simulink model "modello_es_2"  (R2024b)
settings: Solver=VariableStepAuto  StartTime=0.0  StopTime=T  RelTol=1e-3
values from neighbouring files (symbols this model uses):
  b = b_values(i)    [es_2_main.m]
libraries: robotmobilelib x1
settings Model: Creator=feder  LastModifiedBy=feder

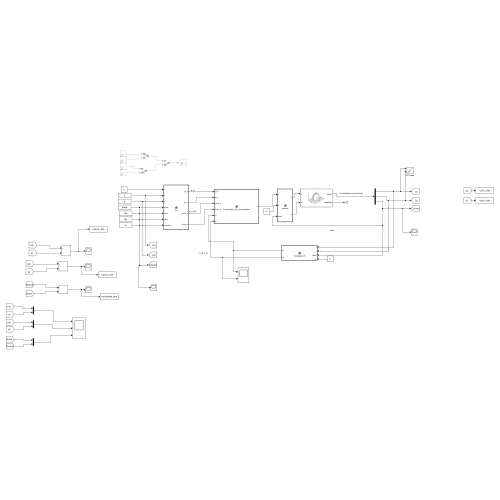
[thumbnail: Simulink's stored preview of the top-level diagram]
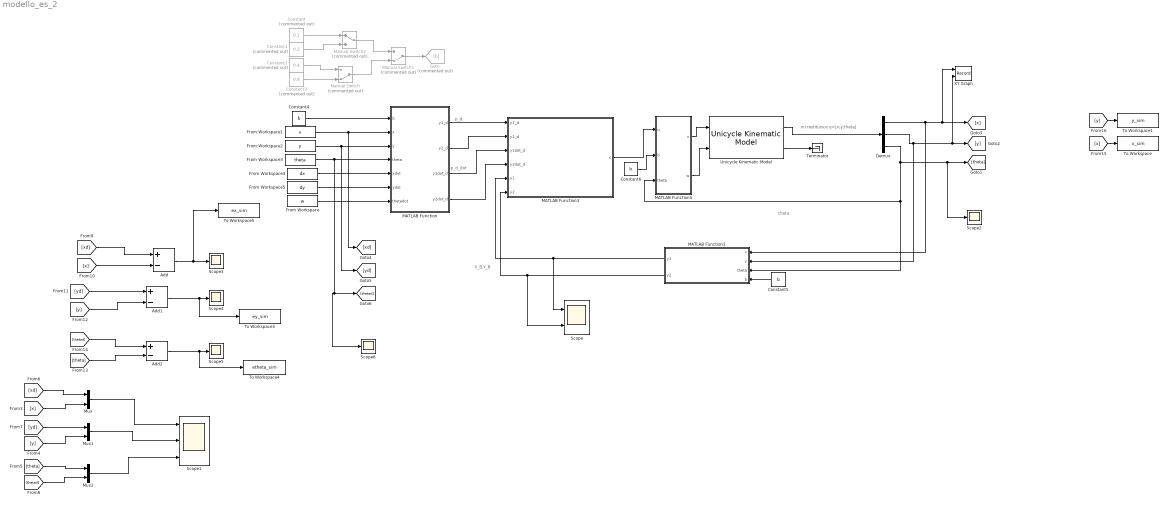
== system modello_es_2 ==
  note: theta
  note: X_B,Y_B
  note: p_d_dot
  note: p_d
  note: mi restituisce q=[x;y;theta]
  Add : Sum  Inputs=+-
  Add1 : Sum  Inputs=+-
  Add2 : Sum  Inputs=+-
  Constant : Constant  Commented=on  Value=0.1
  Constant1 : Constant  Commented=on  Value=0.2
  Constant2 : Constant  Commented=on  Value=0.4
  Constant3 : Constant  Commented=on  Value=0.8
  Constant4 : Constant  Value=b
  Constant5 : Constant  Value=b
  Constant6 : Constant  Value=b
  Demux : Demux  Outputs=3
  From Workspace : FromWorkspace  VariableName=w
  From Workspace1 : FromWorkspace  VariableName=x
  From Workspace2 : FromWorkspace  VariableName=y
  From Workspace3 : FromWorkspace  VariableName=theta
  From Workspace4 : FromWorkspace  VariableName=dx
  From Workspace5 : FromWorkspace  VariableName=dy
  Goto : Goto  Commented=on  GotoTag=b
  MATLAB Function : MATLAB Function  TreatAsAtomicUnit=on
  MATLAB Function2 : MATLAB Function  TreatAsAtomicUnit=on
  MATLAB Function3 : MATLAB Function  TreatAsAtomicUnit=on
  MATLAB Function5 : MATLAB Function  TreatAsAtomicUnit=on
  Manual Switch : ManualSwitch  Commented=on  CurrentSetting=0
  Manual Switch1 : ManualSwitch  Commented=on  CurrentSetting=0
  Manual Switch2 : ManualSwitch  Commented=on
  Mux : Mux  Inputs=2
  Mux1 : Mux  Inputs=2
  Mux2 : Mux  Inputs=2
  Scope : Scope  NumInputPorts=2
  Scope1 : Scope  NumInputPorts=3
  Scope{2..6} (5 alike) : Scope
  Terminator : Terminator
  To Workspace : ToWorkspace  VariableName=x_sim  SaveFormat=Timeseries  SampleTime=-1
  To Workspace1 : ToWorkspace  VariableName=y_sim  SaveFormat=Timeseries  SampleTime=-1
  To Workspace3 : ToWorkspace  VariableName=ey_sim  SaveFormat=Timeseries  SampleTime=-1
  To Workspace4 : ToWorkspace  VariableName=etheta_sim  SaveFormat=Timeseries  SampleTime=-1
  To Workspace5 : ToWorkspace  VariableName=ex_sim  SaveFormat=Timeseries  SampleTime=-1
  Unicycle Kinematic Model : robotmobilelib/Unicycle Kinematic Model  VehicleInputs=Vehicle Speed & Heading Angular Velocity  WheelRadius=0.1  WheelSpeedRange=[-Inf Inf]  InitialState=q_i  SimulateUsing=Interpreted execution
  XY Graph : Record  FileSettingsInternal="{\"entries\":[{\"content\":{\"excelSettings\":{\"content\":{},\"type\":\"Streamout.ExcelSettings\"}},\"type\":\"Streamout.FileSettingStorage\",\"uuid\":\"\"}],\"packageUris\":[\"http:\\/\\/schema.mathworks.com\\/mf0\\/streamout_blocks\\/R2020a\"],\"version\":\"1.0\"}"  Layout=[1 1]  SignalsInternal="{\"entries\":[{\"content\":{\"signals\":[{\"content\":{\"blockPath\":[],\"dimensions\":[1],\"domain\":\"\",\"lineColor\":\"#a2142f\",\"plots\":[ 1 ],\"port\":1,\"sid\":[\"\"],\"signalID\":1,\"signalName\":\"Demux:1\"},\"type\":\"RecordBlkView.Signal\",\"uuid\":\"\"},{\"content\":{\"blockPath\":[],\"dimensions\":[1],\"domain\":\"\",\"lineColor\":\"#139fff\",\"plots\":[ 1 ],\"port\":2,\"sid\":[\"\"],\"signalID\":2,\"signalName\":\"Demux:2\"},\"type\":\"RecordBlkView.Signal\",\"uuid\":\"\"}]},\"type\":\"RecordBlkView.InputSignals\",\"uuid\":\"\"}],\"packageUris\":[\"http:\\/\\/schema.mathworks.com\\/mf0\\/streamout_blocks\\/R2020a\"],\"version\":\"1.0\"}"  VisualizationBindings="{\"xyplotplugin\":{\"info\":[{\"series\":[{\"bindingParametersList\":[{\"parameter\":\"X-Axis\",\"signalID\":1,\"signalName\":\"Demux:1\"},{\"parameter\":\"Y-Axis\",\"signalID\":2,\"signalName\":\"Demux:2\"}],\"seriesID\":0}],\"subplotID\":1}]}}"  CompatibilityTag=XY
  wires:
  From Workspace1/1 -> MATLAB Function/2(x), [xd]
  From Workspace2/1 -> MATLAB Function/3(y), [yd]
  From Workspace4/1 -> MATLAB Function/5(xdot)
  From Workspace5/1 -> MATLAB Function/6(ydot)
  From Workspace/1 -> MATLAB Function/7(thetadot)
  Constant4/1 -> MATLAB Function/1(b)
  Unicycle Kinematic Model/1 -> Demux/1
  Demux/1 -> MATLAB Function2/1(x), XY Graph/1, [x]
  Demux/2 -> MATLAB Function2/2(y), XY Graph/2, [y]
  Demux/3 -> MATLAB Function2/3(theta), MATLAB Function5/3(theta), Scope2/1, [theta]
  [xd] -> Mux/1
  [x] -> Mux/2
  [theta] -> Mux2/1
  [thetad] -> Mux2/2
  [y] -> Mux1/2
  [yd] -> Mux1/1
  Mux2/1 -> Scope1/3
  Mux1/1 -> Scope1/2
  Mux/1 -> Scope1/1
  MATLAB Function/1(y1_d) -> MATLAB Function3/1(y1_d)
  MATLAB Function/2(y2_d) -> MATLAB Function3/2(y2_d)
  MATLAB Function/3(y1dot_d) -> MATLAB Function3/3(y1dot_d)
  MATLAB Function/4(y2dot_d) -> MATLAB Function3/4(y2dot_d)
  [xd] -> Add/1
  [x] -> Add/2
  [yd] -> Add1/1
  [y] -> Add1/2
  [theta] -> Add2/2
  [thetad] -> Add2/1
  Add/1 -> To Workspace5/1, Scope3/1
  Add1/1 -> To Workspace3/1, Scope4/1
  Add2/1 -> To Workspace4/1, Scope5/1
  MATLAB Function2/2(y2) -> MATLAB Function3/6(y2), Scope/2
  MATLAB Function2/1(y1) -> MATLAB Function3/5(y1), Scope/1
  Constant5/1 -> MATLAB Function2/4(b)
  MATLAB Function3/1(u) -> MATLAB Function5/1(u)
  Constant6/1 -> MATLAB Function5/2(b)
  MATLAB Function5/2(w) -> Unicycle Kinematic Model/2
  MATLAB Function5/1(v) -> Unicycle Kinematic Model/1
  Unicycle Kinematic Model/2 -> Terminator/1
  From Workspace3/1 -> [thetad], Scope6/1, MATLAB Function/4(theta)
  Constant3/1 -> Manual Switch/2
  Constant/1 -> Manual Switch2/1
  Manual Switch/1 -> Manual Switch1/2
  Manual Switch1/1 -> Goto/1
  Manual Switch2/1 -> Manual Switch1/1
  Constant1/1 -> Manual Switch2/2
  Constant2/1 -> Manual Switch/1
  [x] -> To Workspace/1
  [y] -> To Workspace1/1

== matlab function modello_es_2/MATLAB Function3 ==
  data: u output; y1_d input; y2_d input; y1dot_d input; y2dot_d input; y1 input; y2 input
function u = ControlLaw_IO_Linearization(y1_d, y2_d, y1dot_d, y2dot_d, y1, y2)

    k1=20;
    k2=15;

    e1 = y1_d - y1;
    e2 = y2_d - y2;

    % Controllo 
    u1 = y1dot_d + k1 * e1;
    u2 = y2dot_d + k2 * e2;

    % Output
    u = [u1; u2];
end

== matlab function modello_es_2/MATLAB Function ==
  data: y1_d output; b input; x input; y input; theta input; xdot input; ydot input; thetadot input; y2_d output; y1dot_d output; y2dot_d output
function [y1_d, y2_d, y1dot_d, y2dot_d] = fcn(b, x, y, theta, xdot, ydot, thetadot)

    %coordinate punto B
    y1_d = x + b * cos(theta);
    y2_d = y + b * sin(theta);

    % Derivate 
    y1dot_d = xdot - b * thetadot * sin(theta);
    y2dot_d = ydot + b * thetadot * cos(theta);

end

== matlab function modello_es_2/MATLAB Function2 ==
  data: x input; y1 output; y input; theta input; b input; y2 output
function [y1,y2] = Compute_B(x,y,theta,b)

    y1 = x + b*cos(theta);
    y2 = y + b*sin(theta);
end

== matlab function modello_es_2/MATLAB Function5 ==
  data: v output; u input; b input; theta input; w output
function [v, w] = inverse(u,b,theta)

    % Matrice T 
    T = [cos(theta), -b * sin(theta);
         sin(theta),  b * cos(theta)];

    % Risoluzione del sistema [v; w] = T^-1 * u
    output = T \ u;
    %output=inv(T)*u;
    % Estrai v e w
    v = output(1);
    w = output(2);
end
